simulink model "sfMediaPlayer"  (R2025b)
settings: Solver=FixedStepDiscrete  StartTime=0.0  StopTime=inf  FixedStep=0.05  RelTol=1e-3  EnableMultiTasking=on
PreLoadFcn:
  | load handel.mat;
  | handel = audioplayer(y,Fs);
  | load chirp.mat;
  | chirp = audioplayer(y,Fs);
  | load train.mat;
  | train = audioplayer(y,Fs);
  | load laughter.mat;
  | laugh = audioplayer(y,Fs);
  | clear y
  | clear Fs
StopFcn:
  | delete(app)
model workspace (MATLAB code in the model file):
  | Ts = 0.01;  % setup system sample rate
undefined symbols (not defined in the file or in its folder): MediaComponentMode, StreamingMode
CloseFcn:
  | clear handel
  | clear chirp
  | clear train
  | clear laugh
  | clear app
settings Model: PacingRate=1.500000  Creator=The MathWorks, Inc.  LastModifiedBy=The MathWorks, Inc.
settings SolverCC: AlgebraicLoopSolver=TrustRegion  MaxZcPerStep=1.0
settings DataIOCC: ExternalInput=TrackName  LimitDataPoints=on  SaveFormat=Array  SaveOutput=off  SaveTime=off  ReturnWorkspaceOutputs=off
settings OptimizationCC: DefaultParameterBehavior=Inlined  ReuseModelBlockBuffer=off  ExpressionDepthLimit=2147483647.0  StateBitsets=on  DataBitsets=on  ZeroExternalMemoryAtStartup=off  ZeroInternalMemoryAtStartup=off  InitFltsAndDblsToZero=on  EfficientFloat2IntCast=on  EfficientMapNaN2IntZero=off  LifeSpan=1  EfficientTunableParamExpr=on
settings DebuggingCC: UnderspecifiedInitializationDetection=Classic  MergeDetectMultiDrivingBlocksExec=none  FcnCallInpInsideContextMsg=warning  UnconnectedInputMsg=warning  UnconnectedOutputMsg=warning  UnconnectedLineMsg=warning  AllowSymbolicDim=off  StateNameClashWarn=warning  SubsystemReferenceDiagnosticForUnitTest=warning  SFUnexpectedBacktrackingDiag=warning  SFNoUnconditionalDefaultTransitionDiag=warning  SFExecutionAtInitializationDiag=none  ArithmeticOperatorsInVariantConditions=warning
settings HardwareCC: ProdBitPerPointer=32.0  ProdBitPerSizeT=32.0  ProdBitPerPtrDiffT=32.0  ProdLargestAtomicFloat=None  ProdWordSize=32.0  ProdHWDeviceType=NEC->V850
settings ModelReferenceCC: EnableRefExpFcnMdlSchedulingChecks=on  ModelReferenceNumInstancesAllowed=Single  PropagateSignalLabelsOutOfModel=off
settings SFSimCC: SimUseLocalCustomCode=off  SimParseCustomCode=off  CustomCodeUndefinedFunction=UseInterfaceOnly
settings RTWCC: SystemTargetFile=ert.tlc  GenCodeOnly=on  TemplateMakefile=ert_default_tmf  GenerateReport=on  RTWUseLocalCustomCode=off  IncludeHyperlinkInReport=on  LaunchReport=on  GenerateTraceInfo=on  GenerateTraceReport=on  GenerateTraceReportSl=on  GenerateTraceReportSf=on  GenerateTraceReportEml=on  GPUComputeCapability=3.5  DLArmComputeVersion=19.05  Description=Real-Time Workshop Embedded Coder (no auto configuration)
settings CodeAppCC: IgnoreCustomStorageClasses=off  CustomSymbolStrType=$N$R$M  CustomSymbolStrModelFcn=$N  StateflowObjectComments=on  InternalIdentifier=Classic
settings ERTTargetCC: InlinedParameterPlacement=Hierarchical  ERTCustomFileTemplate=example_file_process.tlc  ConvertIfToSwitch=off  SuppressUnreachableDefaultCases=off  EnableUserReplacementTypes=on  MultiwordLength=2048.0  GenerateSampleERTMain=on  IncludeMdlTerminateFcn=off  SupportAbsoluteTime=off  PurelyIntegerCode=on  SupportNonFinite=off  SupportComplex=off
settings ConfigComp: CovMetricSettings=dw  CovSaveCumulativeToWorkspaceVar=on  CovSaveSingleToWorkspaceVar=on  CovExternalEMLEnable=off  CovSFcnEnable=off  DVMaxProcessTime=600.0  DVParameters=on  DVModelCoverageObjectives=MCDC  DVMaxTestCaseSteps=500.0  DVTestSuiteOptimization=Auto  DVAbsoluteTolerance=1.0e-5  DVDefectChecker=off  DVDetectActiveLogic=on  DVMaxViolationSteps=20.0  DVHarnessSource=Signal Editor  DVSaveReport=on  DVActiveTab=0.0

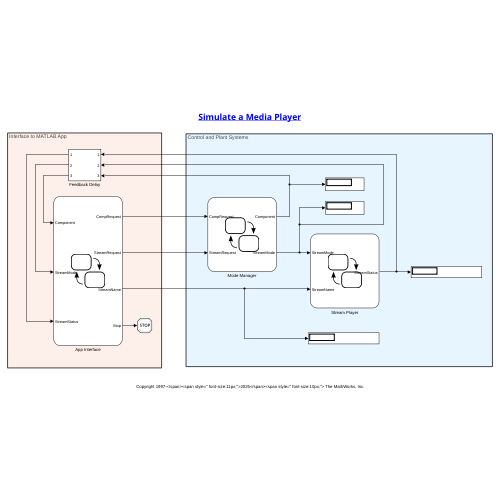
[thumbnail: Simulink's stored preview of the top-level diagram]
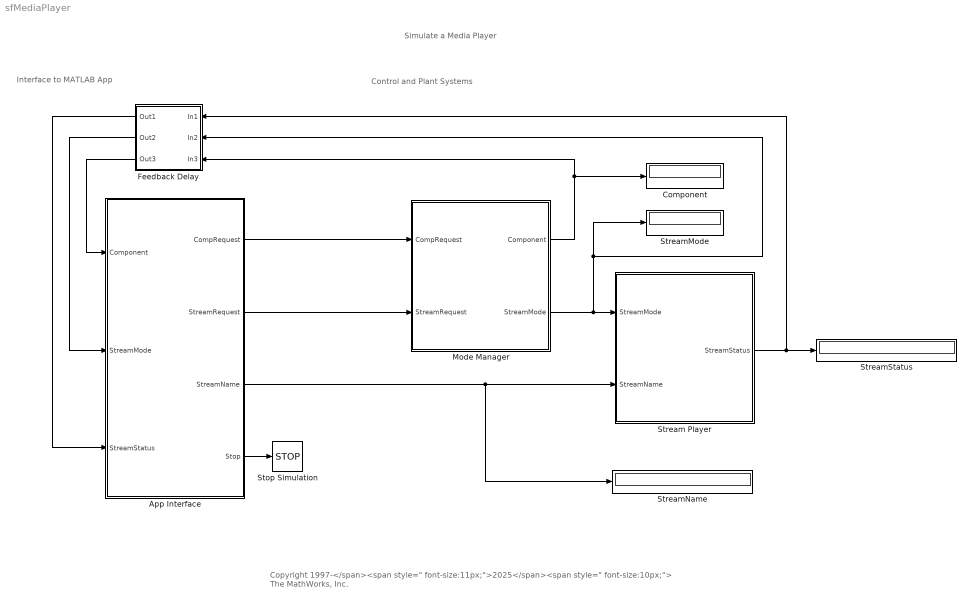
== system sfMediaPlayer ==
  note: Control and Plant Systems
  note: Interface to MATLAB App
  note: Copyright 1997-</span><span style=" font-size:11px;">2025</span><span style=" font-size:10px;"> The MathWorks, Inc.
  note: Simulate a Media Player
  App Interface : Stateflow chart  TreatAsAtomicUnit=on
  Component : Display
  Feedback Delay : Subsystem
  Mode Manager : Stateflow chart  TreatAsAtomicUnit=on
  Stop Simulation : Stop
  Stream Player : Stateflow chart  TreatAsAtomicUnit=on
  StreamMode : Display
  StreamName : Display
  StreamStatus : Display
  wires:
  Mode Manager/2(StreamMode) -> Stream Player/1(StreamMode), Feedback Delay/2(In2), StreamMode/1
  Mode Manager/1(Component) -> Feedback Delay/3(In3), Component/1
  Stream Player/1(StreamStatus) -> Feedback Delay/1(In1), StreamStatus/1
  App Interface/3(StreamName) -> StreamName/1, Stream Player/2(StreamName)
  App Interface/4(Stop) -> Stop Simulation/1
  App Interface/1(CompRequest) -> Mode Manager/1(CompRequest)
  App Interface/2(StreamRequest) -> Mode Manager/2(StreamRequest)
  Feedback Delay/3(Out3) -> App Interface/1(Component)
  Feedback Delay/2(Out2) -> App Interface/2(StreamMode)
  Feedback Delay/1(Out1) -> App Interface/3(StreamStatus)

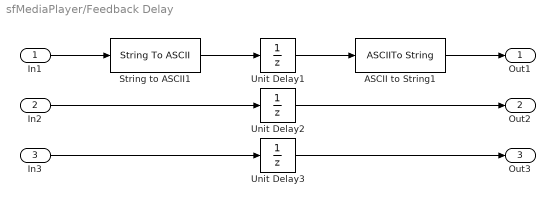
== system sfMediaPlayer/Feedback Delay ==
  In1 : Inport
  In2 : Inport  Port=2
  In3 : Inport  Port=3
  ASCII to String1 : ASCIIToString
  String to ASCII1 : StringToASCII  OutputVectorSize=40
  Unit Delay1 : UnitDelay  SampleTime=-1  HasFrameUpgradeWarning=on
  Unit Delay2 : UnitDelay  InitialCondition=StreamingMode.PLAY  SampleTime=-1  HasFrameUpgradeWarning=on
  Unit Delay3 : UnitDelay  InitialCondition=MediaComponentMode.OFF  SampleTime=-1  HasFrameUpgradeWarning=on
  Out1 : Outport
  Out2 : Outport  Port=2
  Out3 : Outport  Port=3
  wires:
  Unit Delay1/1 -> ASCII to String1/1
  String to ASCII1/1 -> Unit Delay1/1
  ASCII to String1/1 -> Out1/1
  In1/1 -> String to ASCII1/1
  Unit Delay2/1 -> Out2/1
  In2/1 -> Unit Delay2/1
  In3/1 -> Unit Delay3/1
  Unit Delay3/1 -> Out3/1

== stateflow chart sfMediaPlayer/Mode Manager ==
  state Off
    entry:
    Component = OFF;
  state On
    state Stream
      entry:
      Component = STREAM;
      state Pause
        entry:
        StreamMode = PAUSE;
      state Play
        exit:
        StreamMode = PAUSE;
        state Normal
          entry:
          StreamMode = PLAY;
        state Reverse
          entry:
          StreamMode = REW;
        state FastForward
          entry:
          StreamMode = FF;
        (default) -> Normal
        Play -> Normal [order 1] : [StreamRequest == PLAY && !in(Normal)]
        Play -> Reverse [order 2] : [StreamRequest == REW && !in(Reverse)]
        Play -> FastForward [order 3] : [StreamRequest == FF && !in(FastForward)]
      (default) -> Play
      Play -> Pause [order 1] : [StreamRequest == PAUSE]
      Pause -> Play : [StreamRequest == PLAY]
    state Radio
      entry:
      Component = RADIO;
    On -> (junction 181) [order 1] : [hasChanged(CompRequest)]
    (junction 181) -> (junction 127) [order 1] : [CompRequest == RADIO]
    (junction 181) -> Stream [order 2]
    (junction 127) -> Radio
  (default) -> Off
  Off -> (junction 181) : [CompRequest != OFF]
  On -> Off [order 1] : [CompRequest == OFF]
  data: CompRequest input Enum: MediaComponentMode =0xFF; StreamRequest input Enum: StreamingMode; Component output Enum: MediaComponentMode; StreamMode output Enum: StreamingMode

== stateflow chart sfMediaPlayer/App Interface ==
  state InterfaceWithApp
    en:
    CompRequest = OFF;
    StreamRequest = PAUSE;
    StreamName = "";
    Stop = false;
    app = ml.sfMediaPlayerApp(this);
    InterfaceWithApp -> (junction 14)
    (junction 14) -> (junction 16) [order 1] : [hasChanged(Component) || hasChanged(StreamMode)]
    (junction 14) -> (junction 19) [order 2]
    (junction 16) -> (junction 21) : {ml.updateButtons(app);}
    (junction 19) -> (junction 21) [order 1] : [hasChanged(StreamStatus)]
    (junction 19) -> (junction 24) [order 2]
    (junction 21) -> (junction 35) : {ml.updateStatus(app);}
    (junction 24) -> (junction 35)
  (default) -> InterfaceWithApp
  data: CompRequest output Enum: MediaComponentMode; StreamRequest output Enum: StreamingMode; app local ml; Component input Enum: MediaComponentMode; StreamMode input Enum: StreamingMode; StreamName output string; Stop output boolean; StreamStatus input string

== stateflow chart sfMediaPlayer/Stream Player ==
  state Connected
    en:
    N = strlen(StreamName);
    state PLAY
      en:
      StreamStatus = strcat("Playing: ",StreamName);
      state PlaySounds
        state Handel
          en:
          ml.play(ml.handel);
          ex:
          ml.stop(ml.handel);
        state Train
          en:
          ml.play(ml.train);
          ex:
          ml.stop(ml.train);
        state Laugh
          en:
          ml.play(ml.laugh);
          ex:
          ml.stop(ml.laugh);
        state MusicOff
        (default) -> (junction 222) : {i = 0;}
        (junction 222) -> Handel [order 1] : [substr(StreamName,0,6) == "Handel"]
        (junction 222) -> (junction 230) [order 2]
        (junction 230) -> Train [order 1] : [substr(StreamName,0,5) == "Train"]
        (junction 230) -> (junction 232) [order 2]
        (junction 232) -> Laugh [order 1] : [substr(StreamName,0,3) == "Fun"]
        (junction 232) -> (junction 227) [order 2]
        (junction 227) -> MusicOff
    state REW
      en, du:
      StreamStatus = strcat("Reverse << ",substr(StreamName,i,N));
      state UpdateIndex
        en, du: ml.play(ml.chirp);
        ex: ml.stop(ml.chirp);
        state IncModN
        IncModN -> (junction 181) : after(delay,sec){i = i+1;}
        (junction 181) -> (junction 196)
        (junction 196) -> IncModN [order 1] : [i>=N]{i = 0;}
        (junction 196) -> (junction 197) [order 2]
        (junction 197) -> IncModN
    state FF
      en, du:
      StreamStatus = strcat("Forward >> ",substr(StreamName,i,N));
      state UpdateIndex
        en, du: ml.play(ml.chirp);
        ex: ml.stop(ml.chirp);
        state DecModN
        DecModN -> (junction 200) : after(delay,sec){i = i-1;}
        (junction 200) -> (junction 201)
        (junction 201) -> DecModN [order 1] : [i<0]{i = N-1;}
        (junction 201) -> (junction 202) [order 2]
        (junction 202) -> DecModN
    state PAUSE
      en:
      StreamStatus = strcat("Paused: ",StreamName);
    (default) -> (junction 138)
    Connected -> (junction 138) [order 1] : [hasChanged(StreamMode)]
    (junction 138) -> PLAY [order 1] : [StreamMode == PLAY]
    (junction 138) -> (junction 140) [order 2]
    (junction 140) -> REW [order 1] : [StreamMode == REW]
    (junction 140) -> (junction 142) [order 2]
    (junction 142) -> FF [order 1] : [StreamMode == FF]
    (junction 142) -> (junction 144) [order 2]
    (junction 144) -> PAUSE
  state Connecting
    en:
    StreamStatus = strcat("Connecting to ",StreamName);
  (default) -> Connected
  Connected -> Connecting [order 1] : [hasChanged(StreamName)]
  Connecting -> Connected : after(1,sec)
  data: StreamMode input Enum: StreamingMode; StreamStatus output string; StreamName input string; N local int32; i local int32; delay constant double =0.25
